simulink library "casper_library_sources"  (R2021a)
settings: Solver=ode45  StartTime=0.0  StopTime=10.0  RelTol=1e-3
values from neighbouring files (symbols this model uses):
  a = [lenba, lenpa, lenta]    [bus_addsub_init.m]    (also in bus_logical_init.m; bus_maddsub_init.m; bus_mult_init.m; bus_relational_init.m)
  b = [lenbb, lenpb, lentb]    [bus_addsub_init.m]    (also in bus_logical_init.m; bus_maddsub_init.m; bus_mult_init.m; bus_relational_init.m)
libraries: xbsIndex_r4 x11172, $bdroot x2
(part 1 of 29)
settings Model: Creator=mdexter  LastModifiedBy=jkocz
settings SolverCC: AlgebraicLoopSolver=TrustRegion
settings DataIOCC: LimitDataPoints=on  SaveFormat=Array  SignalLoggingSaveFormat=ModelDataLogs  ReturnWorkspaceOutputs=off
settings OptimizationCC: BlockReduction=off  BooleanDataType=off  ExpressionDepthLimit=2147483647  LifeSpan=inf
settings DebuggingCC: SaveWithParameterizedLinksMsg=none  UnderspecifiedInitializationDetection=Classic  MergeDetectMultiDrivingBlocksExec=none  SignalResolutionControl=TryResolveAllWithWarning  FcnCallInpInsideContextMsg=warning  AllowSymbolicDim=off  StateNameClashWarn=warning  SFUnexpectedBacktrackingDiag=warning  SFNoUnconditionalDefaultTransitionDiag=warning  SFExecutionAtInitializationDiag=none  SFMachineParentedDataDiag=warning  ArithmeticOperatorsInVariantConditions=warning
settings HardwareCC: ProdBitPerPointer=32  ProdBitPerSizeT=32  ProdBitPerPtrDiffT=32  ProdLargestAtomicFloat=None  ProdIntDivRoundTo=Undefined  ProdEndianess=Unspecified  ProdWordSize=32  ProdHWDeviceType=32-bit Generic  TargetUnknown=on
settings ModelReferenceCC: PropagateSignalLabelsOutOfModel=off
settings SFSimCC: SimUseLocalCustomCode=off  CustomCodeUndefinedFunction=UseInterfaceOnly
settings RTWCC: RTWUseLocalCustomCode=off
settings CodeAppCC: StateflowObjectComments=on
settings GRTTargetCC: TargetLangStandard=C89/C90 (ANSI)  CombineOutputUpdateFcns=off  GRTInterface=on
settings ConfigComp: CovMetricSettings=dw  CovSaveCumulativeToWorkspaceVar=on  CovSaveSingleToWorkspaceVar=on  CovExternalEMLEnable=off

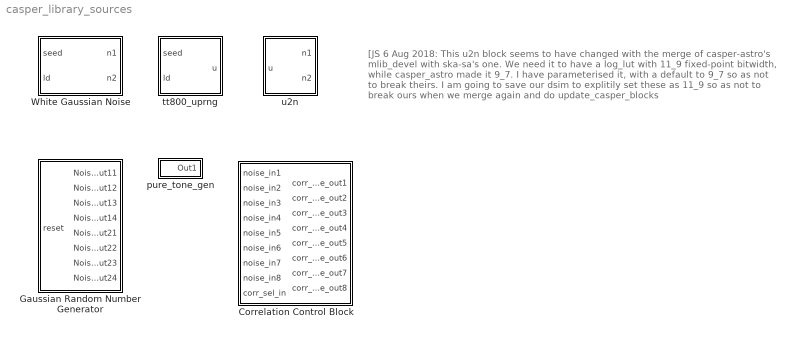
== system casper_library_sources ==
  note: [JS 6 Aug 2018: This u2n block seems to have changed with the merge of
      | casper-astro's mlib_devel with ska-sa's one.
      | We need it to have a log_lut with 11_9 fixed-point bitwidth, while casper_astro
      | made it 9_7. I have parameterised it, with a default to 9_7 so as not to break theirs.
      | I am going to save our dsim to explitily set these as 11_9 so as not to break ours
      | when we merge again and do update_casper_blocks
  Correlation Control Block : Subsystem
      mask help:
      | This block implements a correlation control module.
      | The design possesses an uncorrelation digital noise source
      | whose controlled fraction is added the two inputs to achieve
      | variable correlation at the output.
      | It works with the Gaussian Random Number Generator
      | available in the CASPER library.
  Gaussian Random Number Generator : Subsystem  mask(Gaussian Random Number Generator){}
      mask help:
      | The block contains two uncorrelated Gaussian random
      | number generators (noise sources); each of which
      | has four outputs, thus making it compatible with CASPER correlator
      | designs. This block gives 8-bit two's complement output on each output
      | line. The blocks uses maximal length polynomial sequences combined to
      | give a Gaussian distribution noise (according to the Central
      | Limit Theorem). Reset is synchronous active high.
      mask Help: Please refer to information given inside the subsystems.
  White Gaussian Noise : Subsystem  mask(White Gaussian Noise Generator){seed=hex2dec('32198754'), u2n_log_lut_bitwidth=9, u2n_log_lut_binpoint=7}
      mask help: Outputs two independent white gaussian noise signals as Fix_17_14 values with standard deviation 1.0, expected value 0.0, and crest factor 3.90625 (125/32).
      mask Help:
      | Initial seed is specified by a mask parameter at design time.  Can be reseeded at runtime by applying a UFix_32_0 value on the seed input and pulsing the load port (ld) high for one cycle.  Holding the load port high for more than one cycle is allowed, but it affects the underlying PRNG in undocumented ways.  Drill down into the subsystem if you want to learn more.
      | 
      | This block uses a TT800 uniform pseudo-random number generator followed by a uniform-to-normal converter implementing the Box-Muller Polar algorithm.
      | 
      | The TT800 is a high quality pseudo-random number generator based on a "twisted generialized linear feedback shift register".  Its output sequence repeats after 2^800 samples (~10^240 samples).  For more info see: Matsumoto, M. and Kurita, Y. 1994. "Twisted GFSR generators II", ACM Trans. Model. Comput. Simul. 4, 3 (Jul. 1994), 254-266 (http://doi.acm.org/10.1145/189443.189445).
      mask Callback seed:
      | if str2num(get_param(gcb, 'seed')) == 0
      |     error('Seed cannot be zero.')
      | end
      mask Display:
      | port_label('input',1,'seed');
      | port_label('input',2,'ld');
      | port_label('output',1,'n1');
      | port_label('output',2,'n2');
  pure_tone_gen : Subsystem  mask{adc_demux_factor=8, num_fft_channels=1024, tone_channel=3}
      mask prompts: adc_demux_factor "Number of ADC outputs"; num_fft_channels "Number of FFT channels"; tone_channel "Desired Tone Channel"
  tt800_uprng : Subsystem  mask(TT800 Uniform Psedo-Random Number Generator){seed=hex2dec('12345678')}
      mask help: The TT800 is a high quality pseudo-random number generator based on a "twisted generialized linear feedback shift register". Its output sequence repeats after 2^800 samples (~10^240 samples). For more info see: Matsumoto, M. and Kurita, Y. 1994. "Twisted GFSR generators II", ACM Trans. Model. Comput. Simul. 4, 3 (Jul. 1994), 254-266 (http://doi.acm.org/10.1145/189443.189445).
      mask init:
      | set_param([gcb,'/tt800_seed_gen/LFSR'],'rst_value',sprintf('''%08X''', seed));
      mask Help: Initial seed is specified by a mask parameter at design time.  Can be reseeded at runtime by applying a UFix_32_0 value on the seed input and pulsing the load port (ld) high for one cycle.  Holding the load port high for more than one cycle is allowed, but it affects the generator in undocumented ways.  Drill down into the subsystem if you want to learn more.
      mask Display:
      | port_label('input',1,'seed');
      | port_label('input',2,'ld');
      | port_label('output',1,'u');
  u2n : Subsystem  mask(Uniform to Normal Converter){hideme=off, log_lut_bitwidth=9, log_lut_binpoint=7}
      mask prompts: hideme "Hide me"; log_lut_bitwidth "Log_lut bitwidth"; log_lut_binpoint "Log_lut binary point"
      mask help: Converts a variable with uniform distribution into two independent normally distributed variables.
      mask Help: Converts a variable with uniform distribution into two independent normally distributed variables.

== system casper_library_sources/Correlation Control Block ==
  note: Correlation Control Block version 1.0            12th August, 2011
      | Designed by: Kaushal D. Buch, Digital Back-End Group, Giant Meterwave Radio Telescope, India.
      | For more information / suggestions / feedback, please send email to:
      | kdbuch@gmrt.ncra.tifr.res.in /  kaushal.buch@gmail.com
  note: Note:
      | This block has been designed to work only with the existing "Gaussian Random Number Generator" already
      | available in the CASPER library.
  note: Features:
      | Designed as  an extension to the existing "Gaussian Random Number Generator" in CASPER library.
      | Variable correlation in steps of 0,0.05,0.1,0.2,0.5 and 1.
      | It does not use any specific hardware resources like Block RAMs or multipliers.
      | Both of these can be used individually as noise sources or collectively as two uncorrelated sources.
      | Test Results:
      | This block is tested on a reference POCO design, having 300MHz Bandwidth and 0.89 second integration time.
      | Output power has been made constant irrespective of any mode of correlation.
  note: corr_sel_in selection options:
      | 0 - uncorrelated noise (~0.01)
      | 1- corr coeff 0.05
      | 2 - corr coeff 0.1
      | 3 - corr coeff 0.2
      | 4 - corr coeff 0.5
      | 5 - corr coeff 1
  noise_in1 : Inport
  noise_in2 : Inport  Port=2
  noise_in3 : Inport  Port=3
  noise_in4 : Inport  Port=4
  noise_in5 : Inport  Port=5
  noise_in6 : Inport  Port=6
  noise_in7 : Inport  Port=7
  noise_in8 : Inport  Port=8
  corr_sel_in : Inport  Port=9
  corr_ctrl_blk : Subsystem
      mask help:
      | This block implements a correlation control module.
      | The design possesses an uncorrelation digital noise source
      | whose controlled fraction is added the two inputs to achieve
      | variable correlation at the output.
      | It works with the Gaussian Random Number Generator
      | available in the CASPER library.
      mask Display: plot(xcorr(randn(1024,1)))
  corr_noise_out1 : Outport  VectorParamsAs1DForOutWhenUnconnected=off
  corr_noise_out2 : Outport  Port=2  VectorParamsAs1DForOutWhenUnconnected=off
  corr_noise_out3 : Outport  Port=3  VectorParamsAs1DForOutWhenUnconnected=off
  corr_noise_out4 : Outport  Port=4  VectorParamsAs1DForOutWhenUnconnected=off
  corr_noise_out5 : Outport  Port=5  VectorParamsAs1DForOutWhenUnconnected=off
  corr_noise_out6 : Outport  Port=6  VectorParamsAs1DForOutWhenUnconnected=off
  corr_noise_out7 : Outport  Port=7  VectorParamsAs1DForOutWhenUnconnected=off
  corr_noise_out8 : Outport  Port=8  VectorParamsAs1DForOutWhenUnconnected=off
  wires:
  corr_ctrl_blk/8(corr_noise_out8) -> corr_noise_out8/1
  corr_sel_in/1 -> corr_ctrl_blk/9(corr_sel_in)
  noise_in8/1 -> corr_ctrl_blk/8(noise_in8)
  corr_ctrl_blk/7(corr_noise_out7) -> corr_noise_out7/1
  noise_in7/1 -> corr_ctrl_blk/7(noise_in7)
  corr_ctrl_blk/6(corr_noise_out6) -> corr_noise_out6/1
  noise_in6/1 -> corr_ctrl_blk/6(noise_in6)
  corr_ctrl_blk/5(corr_noise_out5) -> corr_noise_out5/1
  noise_in5/1 -> corr_ctrl_blk/5(noise_in5)
  corr_ctrl_blk/4(corr_noise_out4) -> corr_noise_out4/1
  noise_in4/1 -> corr_ctrl_blk/4(noise_in4)
  corr_ctrl_blk/3(corr_noise_out3) -> corr_noise_out3/1
  noise_in3/1 -> corr_ctrl_blk/3(noise_in3)
  corr_ctrl_blk/2(corr_noise_out2) -> corr_noise_out2/1
  noise_in2/1 -> corr_ctrl_blk/2(noise_in2)
  corr_ctrl_blk/1(corr_noise_out1) -> corr_noise_out1/1
  noise_in1/1 -> corr_ctrl_blk/1(noise_in1)

== system casper_library_sources/Gaussian Random Number Generator ==
  note: Known Limitations:
      | The self powers of both these noise blocks are found to be slightly different.
  note: Features:
      | Each of these outputs have been set to a zero mean.
      | The Kurtosis of each of these sources is around 2.9 to 2.93.
      | Hardware utlization of each of the individual noise blocks is around 2% for Virtex-5 SX95 FPGA.
      | It does not use any specific hardware resources like Block RAMs or multipliers.
      | Both of these can be used individually as noise sources or collectively as two uncorrelated sources.
      | Test Results:
      | This polynomial based noise source is tested on a reference POCO design, at 600MHz ADC clock and 1 second integration time.
      | It has a flat spectrum across all the FFT channels.
      | The normalized cross-correlation of these two noise sources is about 0.001 (integration time: 1 second)
  note: Gaussian Random Number Generator version 1.0             30th October, 2010
      | Designed by: Kaushal D. Buch, Digital Back-End Group, Giant Meterwave Radio Telescope, India.
      | For more information / suggestions / feedback, please send email to:
      | kdbuch@gmrt.ncra.tifr.res.in /  kaushal.buch@gmail.com
  reset : Inport
  Noise Block 1 : Subsystem
      mask Display: plot(randn(1024,1))
  Noise Block 2 : Subsystem
      mask Display: plot(randn(1024,1))
  Noise_Out11 : Outport  VectorParamsAs1DForOutWhenUnconnected=off
  Noise_Out12 : Outport  Port=2  VectorParamsAs1DForOutWhenUnconnected=off
  Noise_Out13 : Outport  Port=3  VectorParamsAs1DForOutWhenUnconnected=off
  Noise_Out14 : Outport  Port=4  VectorParamsAs1DForOutWhenUnconnected=off
  Noise_Out21 : Outport  Port=5  VectorParamsAs1DForOutWhenUnconnected=off
  Noise_Out22 : Outport  Port=6  VectorParamsAs1DForOutWhenUnconnected=off
  Noise_Out23 : Outport  Port=7  VectorParamsAs1DForOutWhenUnconnected=off
  Noise_Out24 : Outport  Port=8  VectorParamsAs1DForOutWhenUnconnected=off
  wires:
  reset/1 -> Noise Block 2/1(reset), Noise Block 1/1(reset)
  Noise Block 2/4(Out4) -> Noise_Out24/1
  Noise Block 2/3(Out3) -> Noise_Out23/1
  Noise Block 2/2(Out2) -> Noise_Out22/1
  Noise Block 2/1(Out1) -> Noise_Out21/1
  Noise Block 1/4(Out4) -> Noise_Out14/1
  Noise Block 1/3(Out3) -> Noise_Out13/1
  Noise Block 1/2(Out2) -> Noise_Out12/1
  Noise Block 1/1(Out1) -> Noise_Out11/1

== system casper_library_sources/White Gaussian Noise ==
  seed : Inport
  ld : Inport  Port=2
  tt800_uprng : $bdroot/tt800_uprng  seed=seed
  u2n : $bdroot/u2n  hideme=off  log_lut_bitwidth=u2n_log_lut_bitwidth  log_lut_binpoint=u2n_log_lut_binpoint
  n1 : Outport  VectorParamsAs1DForOutWhenUnconnected=off
  n2 : Outport  Port=2  VectorParamsAs1DForOutWhenUnconnected=off
  wires:
  tt800_uprng/1 -> u2n/1
  seed/1 -> tt800_uprng/1
  u2n/1 -> n1/1
  ld/1 -> tt800_uprng/2
  u2n/2 -> n2/1

== system casper_library_sources/pure_tone_gen ==
  Sine Wave : Sin  Amplitude=0.9  Frequency=adc_demux_factor*pi/num_fft_channels * tone_channel  SampleTime=1/adc_demux_factor
  Out1 : Outport  VectorParamsAs1DForOutWhenUnconnected=off
  wires:
  Sine Wave/1 -> Out1/1

== system casper_library_sources/tt800_uprng ==
  seed : Inport
  ld : Inport  Port=2
  tt800_engine : Subsystem
  tt800_seed_gen : Subsystem
  u : Outport  VectorParamsAs1DForOutWhenUnconnected=off
  wires:
  ld/1 -> tt800_seed_gen/2(ld)
  tt800_engine/1(u) -> u/1
  seed/1 -> tt800_seed_gen/1(seed_in)
  tt800_seed_gen/2(seed_en) -> tt800_engine/2(seed_en)
  tt800_seed_gen/1(seed_out) -> tt800_engine/1(seed)

== system casper_library_sources/u2n ==
  u : Inport
  Constant2 : xbsIndex_r4/Constant  const=0  gui_display_data_type=Fixed-point  arith_type=Signed (2's comp)  n_bits=8  bin_pt=7  preci_type=Single  exp_width=8  frac_width=24  explicit_period=on  period=1  equ=P=C  opselect=C  inp2=PCIN>>17  opr=+  inp1=P  carry=CIN  dbl_ovrd=off  block_type=constant
  Constant3 : xbsIndex_r4/Constant  const=0  gui_display_data_type=Boolean  arith_type=Boolean  n_bits=16  bin_pt=14  preci_type=Single  exp_width=8  frac_width=24  explicit_period=off  period=1  equ=P=C  opselect=C  inp2=PCIN>>17  opr=+  inp1=P  carry=CIN  dbl_ovrd=off  block_type=constant
  Delay : xbsIndex_r4/Delay  rst=off  infoeditControl=Selection of Reset will increase slice count due to use of real FFs and instead of SRLs  en=off  latency=1  reg_retiming=off  dbl_ovrd=off  block_type=delay
  Delay1 : xbsIndex_r4/Delay  rst=off  infoeditControl=Selection of Reset will increase slice count due to use of real FFs and instead of SRLs  en=off  latency=1  reg_retiming=off  dbl_ovrd=off  block_type=delay
  Delay2 : xbsIndex_r4/Delay  rst=off  infoeditControl=Selection of Reset will increase slice count due to use of real FFs and instead of SRLs  en=off  latency=1  reg_retiming=off  dbl_ovrd=off  block_type=delay
  Gateway Out : xbsIndex_r4/Gateway Out  inherit_from_input=off  hdl_port=off  rows=1  columns=1  UseAsDAC=off  DACChannel='1'  interface=None  automatic_assignment=on  address_offset=hex2dec('00')  intf_name=''  intf_description=''  timing_constraint=None  locs_specified=off  LOCs={}  io_standard={}  block_type=gatewayout
      settings: infoedit="Gateway out block.  Converts Xilinx fixed point inputs into ouputs of type Simulink integer, double, or fixed point.<P><P>Hardware notes:  In hardware these blocks become top level output ports or are discarded, depending on how they are configured."  xl_area=[0 0 0 0 17 0 0]  block_version=10.1.3
  Gateway Out1 : xbsIndex_r4/Gateway Out  inherit_from_input=off  hdl_port=off  rows=1  columns=1  UseAsDAC=off  DACChannel='1'  interface=None  automatic_assignment=on  address_offset=hex2dec('00')  intf_name=''  intf_description=''  timing_constraint=None  locs_specified=off  LOCs={}  io_standard={}  block_type=gatewayout
      settings: infoedit="Gateway out block.  Converts Xilinx fixed point inputs into ouputs of type Simulink integer, double, or fixed point.<P><P>Hardware notes:  In hardware these blocks become top level output ports or are discarded, depending on how they are configured."  xl_area=[0 0 0 0 17 0 0]  block_version=10.1.3
  Scope : Scope  NumInputPorts=2
  bottom_11 : xbsIndex_r4/Slice  nbits=11  boolean_output=off  mode=Lower Bit Location + Width  bit1=0  base1=MSB of Input  bit0=0  base0=LSB of Input  dbl_ovrd=off  block_type=slice
      settings: infoedit="Extracts a given range of bits from each input sample and presents it at the output.  The output type is ordinarily unsigned with binary point at zero, but can be Boolean when the slice is one bit wide.<P><P>Hardware notes: In hardware this block costs nothing."  block_version=10.1.3
  log_lut : xbsIndex_r4/ROM  depth=2^11  initVector=round(2^7*sqrt(-2*log(linspace(2^-11,1,2^11))))/2^7  distributed_mem=Block RAM  rst=off  init_reg=0  en=off  latency=6  gui_display_data_type=Fixed-point  arith_type=Unsigned  n_bits=log_lut_bitwidth  bin_pt=log_lut_binpoint  preci_type=Single  exp_width=8  frac_width=24  optimize=Area  use_rpm=off  dbl_ovrd=off  simulation_type=fast_sim  block_type=sprom
      settings: xl_area=[0 0 1 0 0 0 0]  block_version=10.1.3
  phase_gen : Subsystem
  r_cos : xbsIndex_r4/Mult  precision=Full  arith_type="Signed  (2's comp)"  n_bits=8  bin_pt=2  quantization=Truncate  overflow=Wrap  en=off  latency=3  use_behavioral_HDL=off  opt=Speed  use_embedded=on  optimum_pipeline=off  pipeline=on  dbl_ovrd=off  use_rpm=on  placement_style=Rectangular shape  block_type=mult
      settings: infoedit=Hardware notes: To use the internal pipeline stage of the dedicated multiplier you must select 'Pipeline for maximum performance'.  xl_area=[18 34 0 17 0 1 0]  block_version=10.1.3
  r_sin : xbsIndex_r4/Mult  precision=Full  arith_type="Signed  (2's comp)"  n_bits=8  bin_pt=2  quantization=Truncate  overflow=Wrap  en=off  latency=3  use_behavioral_HDL=off  opt=Speed  use_embedded=on  optimum_pipeline=off  pipeline=on  dbl_ovrd=off  use_rpm=on  placement_style=Rectangular shape  block_type=mult
      settings: infoedit=Hardware notes: To use the internal pipeline stage of the dedicated multiplier you must select 'Pipeline for maximum performance'.  xl_area=[18 34 0 17 0 1 0]  block_version=10.1.3
  sincos_lut : xbsIndex_r4/Dual Port RAM  depth=2^11  initVector=round(128*sin(2*pi*(0:2^11-1)/2^11))/128  distributed_mem=Block RAM  init_a=0  init_b=0  rst_a=off  rst_b=off  en_a=off  en_b=off  latency=1  write_mode_A=Read After Write  write_mode_B=Read After Write  optimize=Area  dbl_ovrd=off  simulation_type=fast_sim  block_type=dpram
  top_11 : xbsIndex_r4/Slice  nbits=11  boolean_output=off  mode=Upper Bit Location + Width  bit1=0  base1=MSB of Input  bit0=0  base0=MSB of Input  dbl_ovrd=off  block_type=slice
      settings: infoedit="Extracts a given range of bits from each input sample and presents it at the output.  The output type is ordinarily unsigned with binary point at zero, but can be Boolean when the slice is one bit wide.<P><P>Hardware notes: In hardware this block costs nothing."  block_version=10.1.3
  n1 : Outport  VectorParamsAs1DForOutWhenUnconnected=off
  n2 : Outport  Port=2  VectorParamsAs1DForOutWhenUnconnected=off
  wires:
  r_cos/1 -> n2/1, Gateway Out1/1
  r_sin/1 -> n1/1, Gateway Out/1
  log_lut/1 -> Delay/1
  u/1 -> bottom_11/1, top_11/1
  top_11/1 -> log_lut/1
  Gateway Out1/1 -> Scope/2
  Gateway Out/1 -> Scope/1
  Delay/1 -> r_cos/1, r_sin/1
  Delay1/1 -> r_sin/2
  Delay2/1 -> r_cos/2
  bottom_11/1 -> phase_gen/1(In1)
  phase_gen/1(ph_sin) -> sincos_lut/1
  sincos_lut/1 -> Delay1/1
  sincos_lut/2 -> Delay2/1
  phase_gen/2(ph_cos) -> sincos_lut/4
  Constant2/1 -> sincos_lut/2, sincos_lut/5
  Constant3/1 -> sincos_lut/3, sincos_lut/6

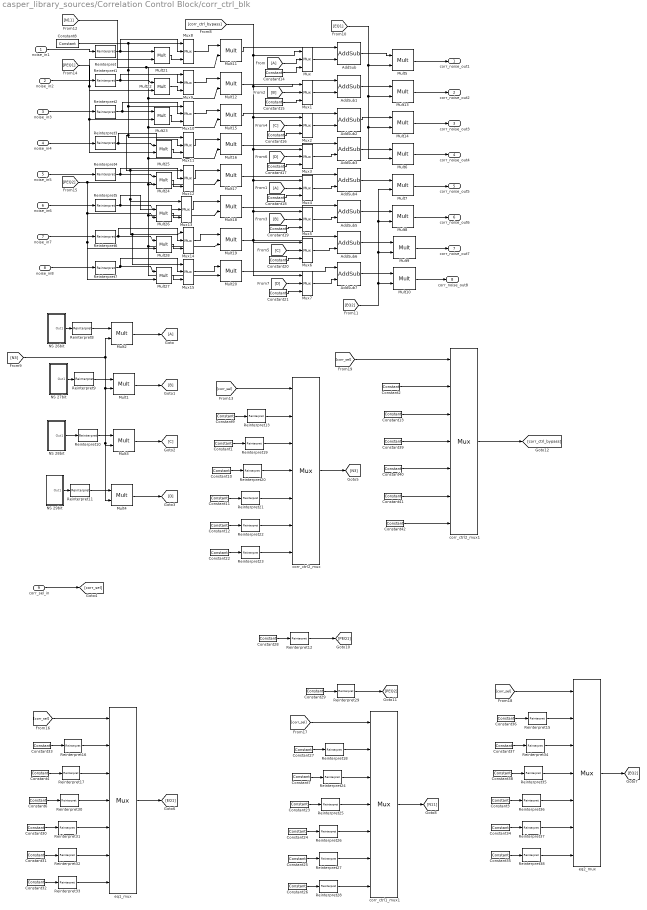
== system casper_library_sources/Correlation Control Block/corr_ctrl_blk ==
  noise_in1 : Inport
  noise_in2 : Inport  Port=2
  noise_in3 : Inport  Port=3
  noise_in4 : Inport  Port=4
  noise_in5 : Inport  Port=5
  noise_in6 : Inport  Port=6
  noise_in7 : Inport  Port=7
  noise_in8 : Inport  Port=8
  corr_sel_in : Inport  Port=9
  AddSub{,1..7} (8 alike) : xbsIndex_r4/AddSub  mode=Addition  use_carryin=off  use_carryout=off  en=off  latency=1  precision=User Defined  arith_type="Signed  (2's comp)"  n_bits=8  bin_pt=7  quantization=Truncate  overflow=Wrap  use_behavioral_HDL=off  hw_selection=Fabric  pipelined=off  use_rpm=on  dbl_ovrd=off  block_type=addsub
      settings: block_version=10.1.3
  Constant1 : xbsIndex_r4/Constant  const=22  gui_display_data_type=Fixed-point  arith_type=Unsigned  n_bits=8  bin_pt=0  preci_type=Single  exp_width=8  frac_width=24  explicit_period=on  period=1  equ=P=C  opselect=C  inp2=PCIN>>17  opr=+  inp1=P  carry=CIN  dbl_ovrd=off  block_type=constant
  Constant10 : xbsIndex_r4/Constant  const=38  gui_display_data_type=Fixed-point  arith_type=Unsigned  n_bits=8  bin_pt=0  preci_type=Single  exp_width=8  frac_width=24  explicit_period=on  period=1  equ=P=C  opselect=C  inp2=PCIN>>17  opr=+  inp1=P  carry=CIN  dbl_ovrd=off  block_type=constant
  Constant11 : xbsIndex_r4/Constant  const=61  gui_display_data_type=Fixed-point  arith_type=Unsigned  n_bits=8  bin_pt=0  preci_type=Single  exp_width=8  frac_width=24  explicit_period=on  period=1  equ=P=C  opselect=C  inp2=PCIN>>17  opr=+  inp1=P  carry=CIN  dbl_ovrd=off  block_type=constant
  Constant12 : xbsIndex_r4/Constant  const=104  gui_display_data_type=Fixed-point  arith_type=Unsigned  n_bits=8  bin_pt=0  preci_type=Single  exp_width=8  frac_width=24  explicit_period=on  period=1  equ=P=C  opselect=C  inp2=PCIN>>17  opr=+  inp1=P  carry=CIN  dbl_ovrd=off  block_type=constant
  Constant{13,39..42} (5 alike) : xbsIndex_r4/Constant  const=0  gui_display_data_type=Fixed-point  arith_type=Boolean  n_bits=8  bin_pt=0  preci_type=Single  exp_width=8  frac_width=24  explicit_period=on  period=1  equ=P=C  opselect=C  inp2=PCIN>>17  opr=+  inp1=P  carry=CIN  dbl_ovrd=off  block_type=constant
  Constant{14..21} (8 alike) : xbsIndex_r4/Constant  const=0  gui_display_data_type=Fixed-point  arith_type=Signed (2's comp)  n_bits=16  bin_pt=8  preci_type=Single  exp_width=8  frac_width=24  explicit_period=on  period=1  equ=P=C  opselect=C  inp2=PCIN>>17  opr=+  inp1=P  carry=CIN  dbl_ovrd=off  block_type=constant
  Constant2 : xbsIndex_r4/Constant  const=1  gui_display_data_type=Fixed-point  arith_type=Boolean  n_bits=8  bin_pt=0  preci_type=Single  exp_width=8  frac_width=24  explicit_period=on  period=1  equ=P=C  opselect=C  inp2=PCIN>>17  opr=+  inp1=P  carry=CIN  dbl_ovrd=off  block_type=constant
  Constant22 : xbsIndex_r4/Constant  const=117  gui_display_data_type=Fixed-point  arith_type=Unsigned  n_bits=8  bin_pt=0  preci_type=Single  exp_width=8  frac_width=24  explicit_period=on  period=1  equ=P=C  opselect=C  inp2=PCIN>>17  opr=+  inp1=P  carry=CIN  dbl_ovrd=off  block_type=constant
  Constant{7,9,23..24,27,29,32..33,36} (9 alike) : xbsIndex_r4/Constant  const=127  gui_display_data_type=Fixed-point  arith_type=Unsigned  n_bits=8  bin_pt=0  preci_type=Single  exp_width=8  frac_width=24  explicit_period=on  period=1  equ=P=C  opselect=C  inp2=PCIN>>17  opr=+  inp1=P  carry=CIN  dbl_ovrd=off  block_type=constant
  Constant25 : xbsIndex_r4/Constant  const=96  gui_display_data_type=Fixed-point  arith_type=Unsigned  n_bits=8  bin_pt=0  preci_type=Single  exp_width=8  frac_width=24  explicit_period=on  period=1  equ=P=C  opselect=C  inp2=PCIN>>17  opr=+  inp1=P  carry=CIN  dbl_ovrd=off  block_type=constant
  Constant26 : xbsIndex_r4/Constant  const=0  gui_display_data_type=Fixed-point  arith_type=Unsigned  n_bits=8  bin_pt=0  preci_type=Single  exp_width=8  frac_width=24  explicit_period=on  period=1  equ=P=C  opselect=C  inp2=PCIN>>17  opr=+  inp1=P  carry=CIN  dbl_ovrd=off  block_type=constant
  Constant28 : xbsIndex_r4/Constant  const=109  gui_display_data_type=Fixed-point  arith_type=Unsigned  n_bits=8  bin_pt=0  preci_type=Single  exp_width=8  frac_width=24  explicit_period=on  period=1  equ=P=C  opselect=C  inp2=PCIN>>17  opr=+  inp1=P  carry=CIN  dbl_ovrd=off  block_type=constant
  Constant3 : xbsIndex_r4/Constant  const=111  gui_display_data_type=Fixed-point  arith_type=Unsigned  n_bits=8  bin_pt=0  preci_type=Single  exp_width=8  frac_width=24  explicit_period=on  period=1  equ=P=C  opselect=C  inp2=PCIN>>17  opr=+  inp1=P  carry=CIN  dbl_ovrd=off  block_type=constant
  Constant30 : xbsIndex_r4/Constant  const=111  gui_display_data_type=Fixed-point  arith_type=Unsigned  n_bits=8  bin_pt=0  preci_type=Single  exp_width=8  frac_width=24  explicit_period=on  period=1  equ=P=C  opselect=C  inp2=PCIN>>17  opr=+  inp1=P  carry=CIN  dbl_ovrd=off  block_type=constant
  Constant31 : xbsIndex_r4/Constant  const=107  gui_display_data_type=Fixed-point  arith_type=Unsigned  n_bits=8  bin_pt=0  preci_type=Single  exp_width=8  frac_width=24  explicit_period=on  period=1  equ=P=C  opselect=C  inp2=PCIN>>17  opr=+  inp1=P  carry=CIN  dbl_ovrd=off  block_type=constant
  Constant34 : xbsIndex_r4/Constant  const=107  gui_display_data_type=Fixed-point  arith_type=Unsigned  n_bits=8  bin_pt=0  preci_type=Single  exp_width=8  frac_width=24  explicit_period=on  period=1  equ=P=C  opselect=C  inp2=PCIN>>17  opr=+  inp1=P  carry=CIN  dbl_ovrd=off  block_type=constant
  Constant35 : xbsIndex_r4/Constant  const=117  gui_display_data_type=Fixed-point  arith_type=Unsigned  n_bits=8  bin_pt=0  preci_type=Single  exp_width=8  frac_width=24  explicit_period=on  period=1  equ=P=C  opselect=C  inp2=PCIN>>17  opr=+  inp1=P  carry=CIN  dbl_ovrd=off  block_type=constant
  Constant37 : xbsIndex_r4/Constant  const=122  gui_display_data_type=Fixed-point  arith_type=Unsigned  n_bits=8  bin_pt=0  preci_type=Single  exp_width=8  frac_width=24  explicit_period=on  period=1  equ=P=C  opselect=C  inp2=PCIN>>17  opr=+  inp1=P  carry=CIN  dbl_ovrd=off  block_type=constant
  Constant38 : xbsIndex_r4/Constant  const=119  gui_display_data_type=Fixed-point  arith_type=Unsigned  n_bits=8  bin_pt=0  preci_type=Single  exp_width=8  frac_width=24  explicit_period=on  period=1  equ=P=C  opselect=C  inp2=PCIN>>17  opr=+  inp1=P  carry=CIN  dbl_ovrd=off  block_type=constant
  Constant4 : xbsIndex_r4/Constant  const=122  gui_display_data_type=Fixed-point  arith_type=Unsigned  n_bits=8  bin_pt=0  preci_type=Single  exp_width=8  frac_width=24  explicit_period=on  period=1  equ=P=C  opselect=C  inp2=PCIN>>17  opr=+  inp1=P  carry=CIN  dbl_ovrd=off  block_type=constant
  Constant6 : xbsIndex_r4/Constant  const=119  gui_display_data_type=Fixed-point  arith_type=Unsigned  n_bits=8  bin_pt=0  preci_type=Single  exp_width=8  frac_width=24  explicit_period=on  period=1  equ=P=C  opselect=C  inp2=PCIN>>17  opr=+  inp1=P  carry=CIN  dbl_ovrd=off  block_type=constant
  Constant8 : xbsIndex_r4/Constant  const=1  gui_display_data_type=Fixed-point  arith_type=Boolean  n_bits=24  bin_pt=0  preci_type=Single  exp_width=8  frac_width=24  explicit_period=on  period=1  equ=P=C  opselect=C  inp2=PCIN>>17  opr=+  inp1=P  carry=CIN  dbl_ovrd=off  block_type=constant
  Mult{1..28} (28 alike) : xbsIndex_r4/Mult  precision=User Defined  arith_type="Signed  (2's comp)"  n_bits=8  bin_pt=7  quantization=Truncate  overflow=Wrap  en=off  latency=3  use_behavioral_HDL=off  opt=Speed  use_embedded=on  optimum_pipeline=off  pipeline=on  dbl_ovrd=off  use_rpm=on  placement_style=Triangular  block_type=mult
      settings: infoedit=Hardware notes: To use the internal pipeline stage of the dedicated multiplier you must select 'Pipeline for maximum performance'.  block_version=10.1.3
  Mux{,1..15} (16 alike) : xbsIndex_r4/Mux  inputs=2  en=off  latency=0  precision=User Defined  arith_type="Signed  (2's comp)"  n_bits=8  bin_pt=7  quantization=Truncate  overflow=Wrap  dbl_ovrd=off  block_type=mux
  NS 26bit : Subsystem  mask(Noise Source Seed Editor){seed1=[0 0 0 1 1 0 0 0 1 0 1 0 0 1 1 1 1 1 1 1 1 1 0 1 0 1], seed2=[1 0 1 1 1 1 1 0 0 1 1 0 0 1 1 0 0 0 0 0 1 1 0 0 1 0], seed3=[0 1 0 1 0 1 0 1 0 1 1 1 1 1 1 0 1 0 1 1 0 1 1 1 1 1], seed4=[0 1 1 0 0 1 1 1 0 0 1 1 0 0 0 0 1 0 0 1 0 0 1 0 1 1], seed5=[1 0 1 1 0 0 1 0 0 0 0 1 1 0 1 1 1 0 0 1 0 0 0 0 1 1], seed6=[0 1 0 0 0 0 0 1 1 1 0 0 0 0 0 1 1 1 1 0 0 0 1 1 1 1], seed7=[1 0 0 0 1 0 0 1 0 0 0 0 1 1 0 0 0 0 1 0 0 0 1 1 0 1], seed8=[1 0 0 1 1 1 0 1 0 1 0 1 1 1 0 1 1 0 0 1 1 0 0 1 0 0], seed9=[0 1 1 1 1 0 0 0 0 0 1 1 1 1 1 0 0 0 0 1 1 1 0 0 0 1], seed10=[0 1 0 0 1 1 1 1 0 0 1 1 1 1 0 0 1 0 0 1 1 1 1 1 0 0], seed11=[0 0 1 0 1 0 1 1 1 0 1 1 0 0 0 0 0 0 1 1 0 0 0 0 0 0], seed12=[1 0 1 1 0 1 1 0 1 0 0 0 1 0 1 0 1 1 0 1 1 0 0 1 0 1], seed13=[1 0 1 0 1 1 0 1 0 0 0 0 1 1 0 1 1 0 0 1 1 0 1 0 0 1], seed14=[1 1 1 1 0 1 0 1 1 0 0 0 1 0 1 1 0 0 0 1 0 0 1 0 0 0]}
      mask prompts: seed1 "Seed 1"; seed2 "Seed 2"; seed3 "Seed 3"; seed4 "Seed 4"; seed5 "Seed 5"; seed6 "Seed 6"; seed7 "Seed 7"; seed8 "Seed 8"; seed9 "Seed 9"; seed10 "Seed 10"; seed11 "Seed 11"; seed12 "Seed 12"; seed13 "Seed 13"; seed14 "Seed 14"
      mask help:
      | Please enter the seed of the polynomials for the noise source.
      | Enter the seed as a row matrix of 1s and 0s. Please ensure to
      | have atleast one '1' in each matrix.
  NS 27bit : Subsystem  mask(Noise Source Seed Editor){seed1=[0 0 1 0 1 1 0 0 0 0 1 0 1 0 0 0 1 1 0 1 1 1 0 0 1 0 1], seed2=[0 1 0 0 1 1 1 0 0 1 1 1 0 1 0 0 0 1 1 1 0 1 1 1 0 1 1], seed3=[0 0 1 0 1 0 0 1 0 0 1 1 1 0 1 0 1 1 1 0 0 0 1 1 0 0 1], seed4=[0 1 0 0 1 0 0 0 1 1 0 0 0 0 0 0 0 0 0 0 1 1 0 1 0 1 1], seed5=[0 0 0 0 0 1 1 0 0 0 0 1 1 1 1 1 0 0 0 1 1 0 0 1 0 1 0], seed6=[1 1 1 0 1 1 0 1 0 0 0 0 1 0 1 0 0 1 1 0 1 1 1 1 1 0 1], seed7=[1 1 1 0 0 1 0 1 0 0 0 0 1 0 0 1 1 0 1 0 0 1 0 0 1 0 1], seed8=[0 0 1 0 0 1 0 0 0 0 1 1 0 0 1 1 0 0 1 0 1 0 1 1 1 1 0], seed9=[0 0 1 1 0 0 1 1 1 1 1 0 0 1 0 1 0 0 0 0 1 1 1 0 1 0 1], seed10=[0 1 1 0 0 0 1 0 1 0 0 1 1 1 1 0 1 1 0 0 1 1 0 1 0 0 0], seed11=[1 1 1 1 0 1 1 1 0 1 1 1 1 0 0 1 1 1 1 1 0 0 1 0 0 0 0], seed12=[1 0 0 0 0 1 0 1 0 1 0 0 1 1 1 1 1 1 1 0 1 0 0 1 1 0 1], seed13=[1 0 1 1 0 1 1 1 1 1 1 1 1 1 1 0 0 1 0 0 0 1 0 1 1 1 0], seed14=[1 0 0 1 1 1 0 0 0 1 1 0 0 0 0 1 0 1 1 1 1 1 1 0 1 1 0]}
      mask prompts: seed1 "Seed 1"; seed2 "Seed 2"; seed3 "Seed 3"; seed4 "Seed 4"; seed5 "Seed 5"; seed6 "Seed 6"; seed7 "Seed 7"; seed8 "Seed 8"; seed9 "Seed 9"; seed10 "Seed 10"; seed11 "Seed 11"; seed12 "Seed 12"; seed13 "Seed 13"; seed14 "Seed 14"
      mask help:
      | Please enter the seed of the polynomials for the noise source.
      | Enter the seed as a row matrix of 1s and 0s. Please ensure to
      | have atleast one '1' in each matrix.
  NS 28bit : Subsystem  mask(Noise Source Seed Editor){seed1=[0 1 0 1 1 0 0 0 1 0 0 1 0 1 0 1 0 0 0 1 0 0 0 1 1 1 1 0], seed2=[0 0 0 0 1 0 1 1 0 0 0 0 0 1 0 1 1 0 0 0 1 1 0 0 0 1 0 1], seed3=[0 1 0 1 1 0 1 0 0 0 1 1 0 0 1 0 1 0 0 0 1 1 1 1 1 1 1 0], seed4=[0 1 0 1 1 1 0 1 0 0 0 0 0 1 0 1 0 1 1 1 1 1 1 0 0 0 1 0], seed5=[0 1 0 0 1 0 0 1 1 0 0 1 1 1 0 1 0 1 1 1 1 0 0 0 0 0 0 0], seed6=[0 0 1 0 1 1 0 0 0 0 0 0 1 1 1 1 1 0 1 1 1 0 1 0 1 1 0 1], seed7=[0 0 0 0 0 1 0 0 0 0 0 1 0 0 0 1 0 1 1 0 1 1 0 1 0 1 1 1], seed8=[0 1 0 0 1 1 1 0 0 1 0 1 1 0 0 1 1 0 0 1 0 1 1 1 1 1 0 1], seed9=[1 1 1 1 1 1 1 0 1 0 0 1 0 0 1 0 0 0 0 0 1 1 1 1 1 1 0 0], seed10=[0 1 1 1 1 1 0 0 1 1 1 1 0 0 1 1 1 1 0 1 1 0 1 0 0 0 0 0], seed11=[1 1 1 1 1 1 1 0 0 1 1 1 1 1 0 0 0 1 1 1 1 0 1 0 1 0 0 0], seed12=[0 0 0 1 0 0 0 1 0 1 1 0 0 1 1 0 1 1 1 0 1 1 1 1 1 0 0 0], seed13=[1 1 0 0 1 0 0 1 0 0 1 0 1 0 0 1 0 1 0 1 1 1 1 0 0 1 1 1], seed14=[0 0 1 0 1 0 0 0 0 1 1 0 0 0 0 0 0 1 1 0 0 1 1 0 0 0 0 1]}
      mask prompts: seed1 "Seed 1"; seed2 "Seed 2"; seed3 "Seed 3"; seed4 "Seed 4"; seed5 "Seed 5"; seed6 "Seed 6"; seed7 "Seed 7"; seed8 "Seed 8"; seed9 "Seed 9"; seed10 "Seed 10"; seed11 "Seed 11"; seed12 "Seed 12"; seed13 "Seed 13"; seed14 "Seed 14"
      mask help:
      | Please enter the seed of the polynomials for the noise source.
      | Enter the seed as a row matrix of 1s and 0s. Please ensure to
      | have atleast one '1' in each matrix.
  NS 29bit : Subsystem  mask(Noise Source Seed Editor){seed1=[0 1 1 1 1 0 1 0 1 1 1 1 1 0 1 1 0 0 0 0 1 1 1 0 0 1 0 1 0], seed2=[0 0 1 0 1 1 0 0 0 0 1 0 1 1 0 1 1 1 0 0 1 1 1 1 1 1 0 0 0], seed3=[0 0 0 1 1 0 0 0 0 0 1 1 0 1 0 1 0 0 1 0 0 0 1 1 1 0 0 0 1], seed4=[0 1 1 1 1 1 0 0 1 1 0 1 1 1 0 1 1 1 1 1 0 0 1 0 1 1 1 1 0], seed5=[1 1 1 1 1 1 1 0 1 1 1 1 0 1 1 1 0 1 1 1 1 0 1 0 0 1 0 0 1], seed6=[1 0 1 0 0 1 0 0 0 0 1 1 1 0 0 0 1 1 1 0 1 1 0 0 0 0 0 0 1], seed7=[0 0 1 0 0 1 0 1 0 0 0 1 0 1 0 1 1 1 1 0 0 1 0 0 1 1 0 0 1], seed8=[1 1 1 0 0 1 0 0 0 0 0 1 0 0 0 1 0 0 1 0 1 0 0 1 0 0 0 1 0], seed9=[1 0 1 0 0 0 0 1 1 1 1 1 0 0 1 1 0 1 0 0 0 1 1 0 0 1 0 1 0], seed10=[0 1 0 1 0 1 0 1 0 1 1 0 1 0 0 1 1 1 0 1 1 1 0 0 1 1 0 0 1], seed11=[1 1 1 0 1 1 1 0 0 1 1 1 1 0 0 0 0 0 1 0 0 1 1 0 0 1 1 1 0], seed12=[0 0 0 1 1 1 0 0 0 1 1 1 1 0 1 1 1 1 0 1 1 1 0 1 1 1 1 0 0], seed13=[1 0 1 1 1 0 0 1 1 1 1 1 1 0 1 0 1 1 0 0 0 1 1 0 0 0 0 1 1], seed14=[1 1 0 0 1 0 0 1 0 1 0 0 0 1 1 1 0 1 1 1 1 0 1 0 0 1 0 1 1]}
      mask prompts: seed1 "Seed 1"; seed2 "Seed 2"; seed3 "Seed 3"; seed4 "Seed 4"; seed5 "Seed 5"; seed6 "Seed 6"; seed7 "Seed 7"; seed8 "Seed 8"; seed9 "Seed 9"; seed10 "Seed 10"; seed11 "Seed 11"; seed12 "Seed 12"; seed13 "Seed 13"; seed14 "Seed 14"
      mask help:
      | Please enter the seed of the polynomials for the noise source.
      | Enter the seed as a row matrix of 1s and 0s. Please ensure to
      | have atleast one '1' in each matrix.
  Reinterpret{,1..13,15..38} (38 alike) : xbsIndex_r4/Reinterpret  force_arith_type=on  arith_type="Signed  (2's comp)"  force_bin_pt=on  bin_pt=7  block_type=reinterpret
      settings: infoedit="Changes signal type without altering the binary representation.   You can changed the signal between signed and unsigned, and relocate the binary point.<P><P>Hardware notes: In hardware this block costs nothing.<P><P>Example:  Suppose the input is 6 bits wide, signed, with 2 fractional bits, and the output is forced to unsigned with 0 fractional bits.  Then an input of -2.0 (1110.00 in binary 2's complement) becomes an output of 56 (111000 in binary)."  block_version=10.1.3
  corr_ctrl1_mux1 : xbsIndex_r4/Mux  inputs=6  en=off  latency=0  precision=User Defined  arith_type="Signed  (2's comp)"  n_bits=8  bin_pt=7  quantization=Truncate  overflow=Wrap  dbl_ovrd=off  block_type=mux
  corr_ctrl2_mux : xbsIndex_r4/Mux  inputs=6  en=off  latency=0  precision=User Defined  arith_type="Signed  (2's comp)"  n_bits=8  bin_pt=7  quantization=Truncate  overflow=Wrap  dbl_ovrd=off  block_type=mux
  corr_ctrl2_mux1 : xbsIndex_r4/Mux  inputs=6  en=off  latency=0  precision=User Defined  arith_type=Unsigned  n_bits=1  bin_pt=0  quantization=Truncate  overflow=Wrap  dbl_ovrd=off  block_type=mux
  eq1_mux : xbsIndex_r4/Mux  inputs=6  en=off  latency=0  precision=User Defined  arith_type="Signed  (2's comp)"  n_bits=8  bin_pt=7  quantization=Truncate  overflow=Wrap  dbl_ovrd=off  block_type=mux
  eq2_mux : xbsIndex_r4/Mux  inputs=6  en=off  latency=0  precision=User Defined  arith_type="Signed  (2's comp)"  n_bits=8  bin_pt=7  quantization=Truncate  overflow=Wrap  dbl_ovrd=off  block_type=mux
  corr_noise_out1 : Outport  VectorParamsAs1DForOutWhenUnconnected=off
  corr_noise_out2 : Outport  Port=2  VectorParamsAs1DForOutWhenUnconnected=off
  corr_noise_out3 : Outport  Port=3  VectorParamsAs1DForOutWhenUnconnected=off
  corr_noise_out4 : Outport  Port=4  VectorParamsAs1DForOutWhenUnconnected=off
  corr_noise_out5 : Outport  Port=5  VectorParamsAs1DForOutWhenUnconnected=off
  corr_noise_out6 : Outport  Port=6  VectorParamsAs1DForOutWhenUnconnected=off
  corr_noise_out7 : Outport  Port=7  VectorParamsAs1DForOutWhenUnconnected=off
  corr_noise_out8 : Outport  Port=8  VectorParamsAs1DForOutWhenUnconnected=off
  wires:
  AddSub/1 -> Mult5/1
  AddSub1/1 -> Mult13/1
  AddSub2/1 -> Mult14/1
  AddSub3/1 -> Mult6/1
  AddSub4/1 -> Mult7/1
  AddSub5/1 -> Mult8/1
  AddSub6/1 -> Mult9/1
  AddSub7/1 -> Mult10/1
  Mux/1 -> AddSub/2
  [A] -> Mux/2
  Constant14/1 -> Mux/3
  Mux1/1 -> AddSub1/2
  [B] -> Mux1/2
  Constant15/1 -> Mux1/3
  Mux2/1 -> AddSub2/2
  [C] -> Mux2/2
  Constant16/1 -> Mux2/3
  Mux3/1 -> AddSub3/2
  [D] -> Mux3/2
  Constant17/1 -> Mux3/3
  [A] -> Mux4/2
  Mux4/1 -> AddSub4/2
  Constant18/1 -> Mux4/3
  Mux5/1 -> AddSub5/2
  [B] -> Mux5/2
  Constant19/1 -> Mux5/3
  Mux6/1 -> AddSub6/2
  [C] -> Mux6/2
  Constant20/1 -> Mux6/3
  [D] -> Mux7/2
  Constant21/1 -> Mux7/3
  Mux7/1 -> AddSub7/2
  [corr_ctrl_bypass] -> Mux/1, Mux7/1, Mux6/1, Mux5/1, Mux4/1, Mux3/1, Mux2/1, Mux1/1
  Mult11/1 -> AddSub/1
  Mult12/1 -> AddSub1/1
  Mult15/1 -> AddSub2/1
  Mult16/1 -> AddSub3/1
  Mult17/1 -> AddSub4/1
  Mult18/1 -> AddSub5/1
  Mult19/1 -> AddSub6/1
  Mult20/1 -> AddSub7/1
  [EQ1] -> Mult6/2, Mult14/2, Mult13/2, Mult5/2
  [EQ2] -> Mult7/2, Mult8/2, Mult9/2, Mult10/2
  [N11] -> Mult18/2, Mult20/2, Mult19/2, Mult17/2, Mult16/2, Mult15/2, Mult12/2, Mult11/2
  Reinterpret/1 -> Mux8/2, Mult21/1
  Reinterpret1/1 -> Mux9/2, Mult22/1
  Reinterpret2/1 -> Mux10/2, Mult23/1
  Reinterpret3/1 -> Mux11/2, Mult25/1
  Reinterpret4/1 -> Mux12/2, Mult24/1
  Reinterpret5/1 -> Mux13/2, Mult26/1
  Reinterpret6/1 -> Mux14/2, Mult28/1
  Reinterpret7/1 -> Mux15/2, Mult27/1
  [PEQ1] -> Mult25/2, Mult23/2, Mult22/2, Mult21/2
  [PEQ2] -> Mult27/2, Mult28/2, Mult26/2, Mult24/2
  Mux8/1 -> Mult11/1
  Mult21/1 -> Mux8/3
  Mux9/1 -> Mult12/1
  Mult22/1 -> Mux9/3
  Mux10/1 -> Mult15/1
  Mult23/1 -> Mux10/3
  Mux11/1 -> Mult16/1
  Mult25/1 -> Mux11/3
  Mux12/1 -> Mult17/1
  Mult24/1 -> Mux12/3
  Mult26/1 -> Mux13/3
  Mux13/1 -> Mult18/1
  Mult28/1 -> Mux14/3
  Mux14/1 -> Mult19/1
  Mult27/1 -> Mux15/3
  Mux15/1 -> Mult20/1
  Constant8/1 -> Mux15/1, Mux14/1, Mux13/1, Mux12/1, Mux11/1, Mux10/1, Mux9/1, Mux8/1
  [N3] -> Mult4/2, Mult3/2, Mult1/2, Mult2/2
  Reinterpret11/1 -> Mult4/1
  Reinterpret10/1 -> Mult3/1
  Reinterpret9/1 -> Mult1/1
  Reinterpret8/1 -> Mult2/1
  Mult4/1 -> [D]
  Mult3/1 -> [C]
  Mult1/1 -> [B]
  Mult2/1 -> [A]
  NS 26bit/1(Out1) -> Reinterpret8/1
  NS 27bit/1(Out1) -> Reinterpret9/1
  NS 28bit/1(Out1) -> Reinterpret10/1
  NS 29bit/1(Out1) -> Reinterpret11/1
  corr_ctrl2_mux1/1 -> [corr_ctrl_bypass]
  Constant41/1 -> corr_ctrl2_mux1/6
  Constant13/1 -> corr_ctrl2_mux1/3
  Constant42/1 -> corr_ctrl2_mux1/7
  Constant40/1 -> corr_ctrl2_mux1/5
  Constant39/1 -> corr_ctrl2_mux1/4
  Constant2/1 -> corr_ctrl2_mux1/2
  [corr_sel] -> corr_ctrl2_mux1/1
  [corr_sel] -> eq2_mux/1
  [corr_sel] -> corr_ctrl1_mux1/1
  [corr_sel] -> eq1_mux/1
  [corr_sel] -> corr_ctrl2_mux/1
  corr_sel_in/1 -> [corr_sel]
  eq2_mux/1 -> [EQ2]
  Constant35/1 -> Reinterpret38/1
  Reinterpret38/1 -> eq2_mux/7
  Constant34/1 -> Reinterpret37/1
  Reinterpret37/1 -> eq2_mux/6
  Constant3/1 -> Reinterpret36/1
  Reinterpret36/1 -> eq2_mux/5
  Constant38/1 -> Reinterpret35/1
  Reinterpret35/1 -> eq2_mux/4
  Constant37/1 -> Reinterpret34/1
  Reinterpret34/1 -> eq2_mux/3
  Constant36/1 -> Reinterpret15/1
  Reinterpret15/1 -> eq2_mux/2
  eq1_mux/1 -> [EQ1]
  Constant32/1 -> Reinterpret33/1
  Reinterpret33/1 -> eq1_mux/7
  Constant31/1 -> Reinterpret32/1
  Reinterpret32/1 -> eq1_mux/6
  Constant30/1 -> Reinterpret31/1
  Reinterpret31/1 -> eq1_mux/5
  Constant6/1 -> Reinterpret30/1
  Reinterpret30/1 -> eq1_mux/4
  Constant4/1 -> Reinterpret17/1
  Reinterpret17/1 -> eq1_mux/3
  Constant33/1 -> Reinterpret16/1
  Reinterpret16/1 -> eq1_mux/2
  Constant29/1 -> Reinterpret29/1
  Reinterpret29/1 -> [PEQ2]
  Constant28/1 -> Reinterpret12/1
  Reinterpret12/1 -> [PEQ1]
  corr_ctrl1_mux1/1 -> [N11]
  Constant26/1 -> Reinterpret28/1
  Reinterpret28/1 -> corr_ctrl1_mux1/7
  Constant25/1 -> Reinterpret27/1
  Reinterpret27/1 -> corr_ctrl1_mux1/6
  Constant24/1 -> Reinterpret26/1
  Reinterpret26/1 -> corr_ctrl1_mux1/5
  Constant23/1 -> Reinterpret25/1
  Reinterpret25/1 -> corr_ctrl1_mux1/4
  Constant7/1 -> Reinterpret24/1
  Reinterpret24/1 -> corr_ctrl1_mux1/3
  Constant27/1 -> Reinterpret18/1
  Reinterpret18/1 -> corr_ctrl1_mux1/2
  corr_ctrl2_mux/1 -> [N3]
  Constant22/1 -> Reinterpret23/1
  Reinterpret23/1 -> corr_ctrl2_mux/7
  Constant12/1 -> Reinterpret22/1
  Reinterpret22/1 -> corr_ctrl2_mux/6
  Constant11/1 -> Reinterpret21/1
  Reinterpret21/1 -> corr_ctrl2_mux/5
  Constant10/1 -> Reinterpret20/1
  Reinterpret20/1 -> corr_ctrl2_mux/4
  Constant1/1 -> Reinterpret19/1
  Reinterpret19/1 -> corr_ctrl2_mux/3
  Constant9/1 -> Reinterpret13/1
  Reinterpret13/1 -> corr_ctrl2_mux/2
  Mult10/1 -> corr_noise_out8/1
  Mult9/1 -> corr_noise_out7/1
  Mult8/1 -> corr_noise_out6/1
  Mult7/1 -> corr_noise_out5/1
  Mult6/1 -> corr_noise_out4/1
  Mult14/1 -> corr_noise_out3/1
  Mult13/1 -> corr_noise_out2/1
  Mult5/1 -> corr_noise_out1/1
  noise_in8/1 -> Reinterpret7/1
  noise_in7/1 -> Reinterpret6/1
  noise_in6/1 -> Reinterpret5/1
  noise_in5/1 -> Reinterpret4/1
  noise_in4/1 -> Reinterpret3/1
  noise_in3/1 -> Reinterpret2/1
  noise_in2/1 -> Reinterpret1/1
  noise_in1/1 -> Reinterpret/1

== system casper_library_sources/Gaussian Random Number Generator/Noise Block 1 ==
  note: The seeds of the individual noise sources can be changed. But the seeds need to be mutually uncorrelated for a particular source
      | i.e. considering only one source say Noise Source -1 ,all the fourteen seeds within that source have to mutually uncorrelated.
  reset : Inport
  Noise Source - 1 : Subsystem  mask(Noise Source Seed Editor){seed1=[0 0 1 0 0 0 0 0 0 1 0 0 1 1 0 0 0 0], seed2=[0 0 0 0 0 0 1 0 1 1 0 0 1 1 0 1 1 1], seed3=[1 0 1 0 0 0 1 0 0 1 0 0 0 0 1 1 0 1], seed4=[1 0 0 0 1 0 0 1 1 0 1 0 0 1 1 0 1 1], seed5=[0 0 1 1 0 1 0 1 1 0 1 1 0 1 0 0 1 0], seed6=[0 1 0 1 0 0 0 0 1 1 1 0 1 0 1 0 1 0], seed7=[0 0 1 0 1 1 0 1 1 0 0 0 0 0 0 0 1 0], seed8=[0 0 1 1 1 1 0 0 1 1 0 0 1 1 0 1 1 1], seed9=[0 1 1 0 0 1 1 0 0 0 0 1 1 1 1 1 0 0], seed10=[0 1 1 0 1 1 1 1 0 0 0 1 0 0 1 1 1 1], seed11=[0 0 0 1 0 0 0 1 0 1 1 1 0 0 0 1 0 0], seed12=[0 1 1 1 1 0 0 0 0 1 1 0 0 1 1 1 0 1], seed13=[0 1 1 1 0 0 1 1 0 0 0 1 1 0 0 0 0 1], seed14=[1 0 0 0 1 1 0 1 0 1 1 1 1 1 1 0 1 0]}
      mask prompts: seed1 "Seed 1"; seed2 "Seed 2"; seed3 "Seed 3"; seed4 "Seed 4"; seed5 "Seed 5"; seed6 "Seed 6"; seed7 "Seed 7"; seed8 "Seed 8"; seed9 "Seed 9"; seed10 "Seed 10"; seed11 "Seed 11"; seed12 "Seed 12"; seed13 "Seed 13"; seed14 "Seed 14"
      mask help:
      | Please enter the seed of the polynomials for the noise source.
      | Enter the seed as a row matrix of 1s and 0s. Please ensure to
      | have atleast one '1' in each matrix.
  Noise Source - 2 : Subsystem  mask(Noise Source Seed Editor){seed1=[1 1 1 1 1 0 1 0 0 0 1 0 0 1 1 0 1 1 0], seed2=[0 1 0 0 1 0 1 1 1 1 1 1 0 0 0 1 1 1 0], seed3=[0 0 1 0 0 1 1 1 0 0 0 1 0 0 0 1 1 1 1], seed4=[1 0 1 0 1 1 0 0 1 0 1 1 0 1 1 0 1 1 1], seed5=[1 0 0 1 1 0 0 0 0 1 0 1 1 1 0 0 1 0 1], seed6=[1 0 1 1 0 0 0 0 1 1 1 0 1 0 0 0 1 0 0], seed7=[1 1 0 1 0 0 1 0 1 1 0 0 0 0 1 0 1 1 0], seed8=[0 0 1 0 1 0 1 1 1 0 1 1 1 1 0 0 0 0 0], seed9=[1 0 1 1 1 1 1 1 0 1 0 0 1 0 1 0 1 1 0], seed10=[1 0 1 0 1 0 0 1 1 0 0 1 0 1 0 0 1 0 1], seed11=[1 1 1 1 0 0 0 1 1 1 0 0 1 1 0 1 1 1 0], seed12=[0 1 0 0 0 1 1 1 0 1 0 0 0 1 0 1 1 0 0], seed13=[0 1 1 0 1 0 0 1 0 0 0 1 0 0 0 1 1 1 0], seed14=[0 1 0 1 1 0 1 0 1 1 0 0 1 1 1 0 1 1 1]}
      mask prompts: seed1 "Seed 1"; seed2 "Seed 2"; seed3 "Seed 3"; seed4 "Seed 4"; seed5 "Seed 5"; seed6 "Seed 6"; seed7 "Seed 7"; seed8 "Seed 8"; seed9 "Seed 9"; seed10 "Seed 10"; seed11 "Seed 11"; seed12 "Seed 12"; seed13 "Seed 13"; seed14 "Seed 14"
      mask help:
      | Please enter the seed of the polynomials for the noise source.
      | Enter the seed as a row matrix of 1s and 0s. Please ensure to
      | have atleast one '1' in each matrix.
  Noise Source - 3 : Subsystem  mask(Noise Source Seed Editor){seed1=[0 0 1 0 1 0 0 0 1 1 1 0 0 0 1 0 1 0 0 0], seed2=[1 1 0 0 0 1 0 0 1 1 1 0 0 0 0 1 0 0 0 0], seed3=[1 1 1 0 1 0 0 1 1 0 0 1 1 1 1 1 1 0 1 0], seed4=[1 0 0 0 1 1 1 1 1 0 0 1 1 1 1 0 0 1 1 0], seed5=[1 0 0 1 0 0 1 0 1 0 0 1 0 0 0 1 1 0 0 1], seed6=[0 1 1 1 1 0 0 1 0 1 0 0 1 1 0 1 1 0 0 1], seed7=[0 1 1 0 0 1 0 0 1 1 1 1 0 0 1 1 0 0 0 1], seed8=[0 1 1 1 0 1 1 1 1 1 0 1 1 1 0 0 1 1 1 0], seed9=[0 1 0 0 1 1 0 0 1 1 1 0 1 0 0 0 0 0 0 0], seed10=[0 1 1 1 1 0 1 1 1 0 0 1 1 1 0 1 0 0 0 0], seed11=[0 0 0 1 0 0 1 0 1 1 0 1 1 1 0 1 0 1 1 0], seed12=[1 1 1 1 1 1 1 0 1 0 0 0 0 1 0 0 0 0 1 0], seed13=[0 0 1 0 1 0 1 1 1 1 0 1 1 1 1 1 1 0 0 0], seed14=[0 1 0 1 0 0 0 1 1 1 1 1 1 1 1 1 1 0 0 1]}
      mask prompts: seed1 "Seed 1"; seed2 "Seed 2"; seed3 "Seed 3"; seed4 "Seed 4"; seed5 "Seed 5"; seed6 "Seed 6"; seed7 "Seed 7"; seed8 "Seed 8"; seed9 "Seed 9"; seed10 "Seed 10"; seed11 "Seed 11"; seed12 "Seed 12"; seed13 "Seed 13"; seed14 "Seed 14"
      mask help:
      | Please enter the seed of the polynomials for the noise source.
      | Enter the seed as a row matrix of 1s and 0s. Please ensure to
      | have atleast one '1' in each matrix.
  Noise Source - 4 : Subsystem  mask(Noise Source Seed Editor){seed1=[1 0 1 0 1 0 1 0 0 1 0 0 1 0 1 1 1 0 1 0 0], seed2=[1 1 1 1 1 0 0 0 1 1 0 0 1 1 1 0 0 0 0 1 0], seed3=[0 1 1 0 0 0 0 1 0 0 1 1 1 1 0 1 1 1 0 1 1], seed4=[1 1 1 1 0 1 0 0 1 1 0 1 1 1 1 1 1 1 0 0 0], seed5=[1 1 1 1 0 1 0 0 1 1 0 1 1 1 1 1 1 1 0 0 0], seed6=[1 0 1 0 1 0 1 0 1 1 0 0 1 1 1 1 0 0 0 1 1], seed7=[1 1 0 1 1 0 0 1 1 1 0 1 1 0 1 1 0 1 0 0 0], seed8=[1 1 0 0 1 1 1 0 0 0 0 1 1 0 0 1 1 1 0 1 1], seed9=[1 0 0 0 0 0 1 0 0 0 1 0 0 1 1 0 1 0 1 1 0], seed10=[1 1 0 1 0 1 1 0 0 1 0 0 1 1 0 0 1 1 1 1 0], seed11=[1 0 0 1 1 1 1 0 1 0 0 1 1 1 0 1 0 0 1 0 1], seed12=[1 0 0 0 1 1 0 1 1 0 1 1 0 1 1 1 0 0 1 0 0], seed13=[1 1 0 1 0 1 0 0 0 1 1 1 1 1 0 1 0 1 0 1 0], seed14=[1 0 1 0 1 1 1 0 0 0 1 1 0 0 1 0 1 0 0 0 1]}
      mask prompts: seed1 "Seed 1"; seed2 "Seed 2"; seed3 "Seed 3"; seed4 "Seed 4"; seed5 "Seed 5"; seed6 "Seed 6"; seed7 "Seed 7"; seed8 "Seed 8"; seed9 "Seed 9"; seed10 "Seed 10"; seed11 "Seed 11"; seed12 "Seed 12"; seed13 "Seed 13"; seed14 "Seed 14"
      mask help:
      | Please enter the seed of the polynomials for the noise source.
      | Enter the seed as a row matrix of 1s and 0s. Please ensure to
      | have atleast one '1' in each matrix.
  Out1 : Outport  VectorParamsAs1DForOutWhenUnconnected=off
  Out2 : Outport  Port=2  VectorParamsAs1DForOutWhenUnconnected=off
  Out3 : Outport  Port=3  VectorParamsAs1DForOutWhenUnconnected=off
  Out4 : Outport  Port=4  VectorParamsAs1DForOutWhenUnconnected=off
  wires:
  reset/1 -> Noise Source - 4/1(reset), Noise Source - 3/1(reset), Noise Source - 2/1(reset), Noise Source - 1/1(reset)
  Noise Source - 4/1(Out1) -> Out4/1
  Noise Source - 3/1(Out1) -> Out3/1
  Noise Source - 2/1(Out1) -> Out2/1
  Noise Source - 1/1(Out1) -> Out1/1
